simulink model "test_SimulinkMdl2_qLPVMPCbeta"  (R2023a)
settings: Solver=FixedStepAuto  StartTime=0.0  StopTime=400  FixedStep=DT  RelTol=1e-3
values from neighbouring files (symbols this model uses):
  DT = 0.008    [dataDLR.m]    (also in generateReport.m; initLPVParam.m; initWorkspace.m; runCalculateEvalCriteria.m)
  Lin_points : value not decoded    [DD_test.sldd]
undefined symbols (not defined in the file or in its folder): Rotor_Lambda
settings Model: DataDictionary=DD_test.sldd  ExtModeTrigMode=oneshot  Creator=Hazim Namik  LastModifiedBy=ditt_aj
settings SolverCC: AlgebraicLoopSolver=TrustRegion
settings DataIOCC: LimitDataPoints=on  SaveFormat=Array  ReturnWorkspaceOutputs=off
settings OptimizationCC: BlockReduction=off  BooleanDataType=off  LifeSpan=inf
settings DebuggingCC: SaveWithParameterizedLinksMsg=none  UnderspecifiedInitializationDetection=Classic  MergeDetectMultiDrivingBlocksExec=none  SignalResolutionControl=TryResolveAllWithWarning  UnconnectedInputMsg=warning  UnconnectedOutputMsg=warning  UnconnectedLineMsg=warning  SFUnexpectedBacktrackingDiag=warning  SFNoUnconditionalDefaultTransitionDiag=warning  SFExecutionAtInitializationDiag=none  ArithmeticOperatorsInVariantConditions=warning
settings HardwareCC: ProdBitPerPointer=32  ProdBitPerSizeT=32  ProdBitPerPtrDiffT=32  ProdLargestAtomicFloat=None  ProdIntDivRoundTo=Undefined  ProdEndianess=Unspecified  ProdWordSize=32  ProdHWDeviceType=32-bit Generic  TargetUnknown=on
settings ModelReferenceCC: EnableRefExpFcnMdlSchedulingChecks=on  PropagateSignalLabelsOutOfModel=off
settings SFSimCC: SimUseLocalCustomCode=off  CustomCodeUndefinedFunction=UseInterfaceOnly
settings RTWCC: RTWUseLocalCustomCode=off  DLArmComputeVersion=19.05
settings CodeAppCC: StateflowObjectComments=on
settings GRTTargetCC: TargetLangStandard=C89/C90 (ANSI)
settings ConfigComp: CovMetricSettings=dw  CovSaveCumulativeToWorkspaceVar=on  CovSaveSingleToWorkspaceVar=on  CovExternalEMLEnable=off

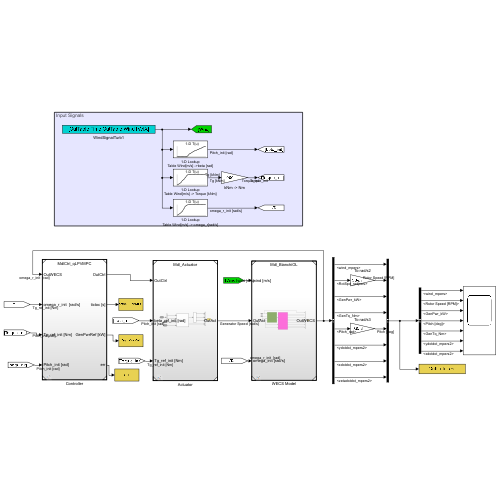
[thumbnail: Simulink's stored preview of the top-level diagram]
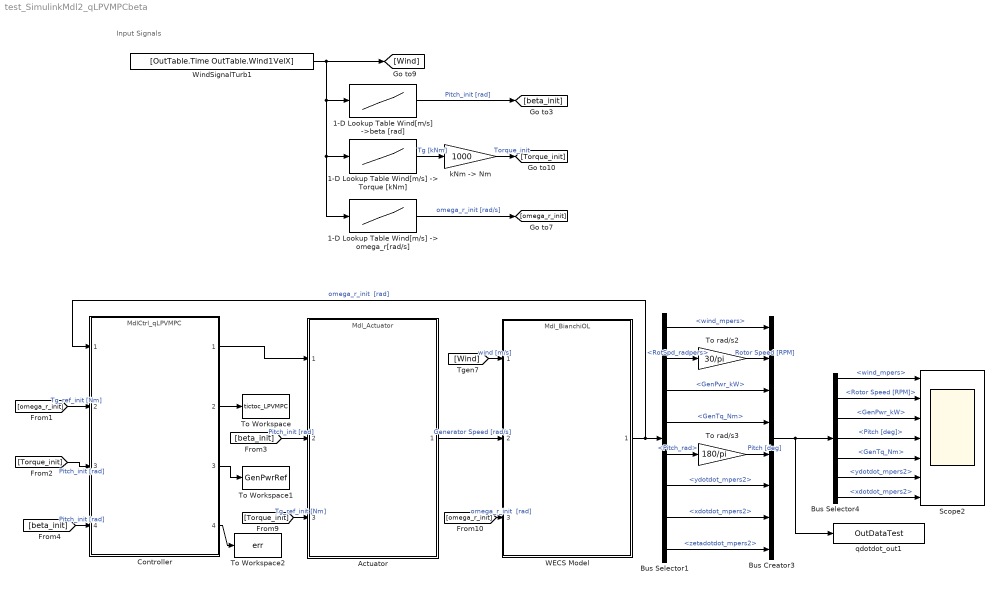
== system test_SimulinkMdl2_qLPVMPCbeta ==
  note: Input Signals
  "1-D Lookup Table Wind[m/s] -> Torque [kNm]" : Lookup_n-D  NumberOfTableDimensions=1  BreakpointsForDimension1=Lin_points.V  BreakpointsForDimension2=Rotor_Lambda  Table=Lin_points.Torque  InternalRulePriority=Speed  RndMeth=Simplest
  "1-D Lookup Table Wind[m/s] -> omega_r[rad/s]" : Lookup_n-D  NumberOfTableDimensions=1  BreakpointsForDimension1=Lin_points.V  BreakpointsForDimension2=Rotor_Lambda  Table=Lin_points.RSpeed  InternalRulePriority=Speed  RndMeth=Simplest
  1-D Lookup Table Wind[m/s] ->beta [rad] : Lookup_n-D  NumberOfTableDimensions=1  BreakpointsForDimension1=Lin_points.V  BreakpointsForDimension2=Rotor_Lambda  Table=Lin_points.Pitch  InternalRulePriority=Speed  RndMeth=Simplest
  Actuator : ModelReference  ModelNameDialog=Mdl_Actuator.slx  SimulationMode=Normal  ModelReferenceVersion=7.0
  Bus Creator3 : BusCreator  Inputs=8
  Bus Selector1 : BusSelector  OutputSignals=wind_mpers,RotSpd_radpers,GenPwr_kW,GenTq_Nm,Pitch_rad,ydotdot_mpers2,xdotdot_mpers2,zetadotdot_mpers2
  Bus Selector4 : BusSelector  OutputSignals=wind_mpers,Rotor Speed [RPM],GenPwr_kW,Pitch [deg],GenTq_Nm,ydotdot_mpers2,xdotdot_mpers2
  Controller : ModelReference  ModelNameDialog=MdlCtrl_qLPVMPC.slx  SimulationMode=Normal  ModelReferenceVersion=7.38
  Scope2 : Scope  NumInputPorts=7
      settings: Tag=Scope
  To Workspace : ToWorkspace  VariableName=tictoc_LPVMPC  SaveFormat=Timeseries  SampleTime=-1
  To Workspace1 : ToWorkspace  VariableName=GenPwrRef  SaveFormat=Timeseries  SampleTime=-1
  To Workspace2 : ToWorkspace  VariableName=err  SaveFormat=Timeseries  SampleTime=-1
  To rad/s2 : Gain  Gain=30/pi
  To rad/s3 : Gain  Gain=180/pi
  WECS Model : ModelReference  ModelNameDialog=Mdl_BianchiOL.slx  SimulationMode=Normal  ModelReferenceVersion=7.1
  WindSignalTurb1 : FromWorkspace  VariableName=[OutTable.Time OutTable.Wind1VelX]  SampleTime=DT  OutputAfterFinalValue=Holding final value
  "kNm -> Nm" : Gain  Gain=1000
  qdotdot_out1 : ToWorkspace  VariableName=OutDataTest  SampleTime=-1
  wires:
  [Torque_init] -> Controller/3  "Pitch_init [rad]"
  WindSignalTurb1/1 -> [Wind], "1-D Lookup Table Wind[m/s] -> omega_r[rad/s]"/1, "1-D Lookup Table Wind[m/s] -> Torque [kNm]"/1, 1-D Lookup Table Wind[m/s] ->beta [rad]/1
  "kNm -> Nm"/1 -> [Torque_init]  "Torque_init"
  [omega_r_init] -> Controller/2  "Tg_ref_init [Nm]"
  "1-D Lookup Table Wind[m/s] -> omega_r[rad/s]"/1 -> [omega_r_init]  "omega_r_init [rad/s]"
  [Wind] -> WECS Model/1  "wind [m/s]"
  1-D Lookup Table Wind[m/s] ->beta [rad]/1 -> [beta_init]  "Pitch_init [rad]"
  "1-D Lookup Table Wind[m/s] -> Torque [kNm]"/1 -> "kNm -> Nm"/1  "Tg [kNm]"
  [Torque_init] -> Actuator/3  "Tg_ref_init [Nm]"
  Actuator/1 -> WECS Model/2  "Generator Speed [rad/s]"
  [omega_r_init] -> WECS Model/3  "omega_r_init  [rad]"
  Controller/3 -> To Workspace1/1
  [beta_init] -> Actuator/2  "Pitch_init [rad]"
  Bus Selector1/5 -> To rad/s3/1  "<Pitch_rad>"
  To rad/s2/1 -> Bus Creator3/2  "Rotor Speed [RPM]"
  Bus Creator3/1 -> qdotdot_out1/1, Bus Selector4/1
  Bus Selector4/4 -> Scope2/4  "<Pitch [deg]>"
  Bus Selector4/7 -> Scope2/7  "<xdotdot_mpers2>"
  Bus Selector4/6 -> Scope2/6  "<ydotdot_mpers2>"
  Bus Selector4/1 -> Scope2/1  "<wind_mpers>"
  To rad/s3/1 -> Bus Creator3/5  "Pitch [deg]"
  Bus Selector4/5 -> Scope2/5  "<GenTq_Nm>"
  Bus Selector1/2 -> To rad/s2/1  "<RotSpd_radpers>"
  Bus Selector1/1 -> Bus Creator3/1  "<wind_mpers>"
  Bus Selector1/4 -> Bus Creator3/4  "<GenTq_Nm>"
  Bus Selector1/3 -> Bus Creator3/3  "<GenPwr_kW>"
  Bus Selector1/7 -> Bus Creator3/7  "<xdotdot_mpers2>"
  Bus Selector1/6 -> Bus Creator3/6  "<ydotdot_mpers2>"
  Bus Selector4/3 -> Scope2/3  "<GenPwr_kW>"
  Bus Selector4/2 -> Scope2/2  "<Rotor Speed [RPM]>"
  WECS Model/1 -> Controller/1, Bus Selector1/1  "omega_r_init  [rad]"
  [beta_init] -> Controller/4  "Pitch_init [rad]"
  Controller/1 -> Actuator/1
  Controller/2 -> To Workspace/1
  Controller/4 -> To Workspace2/1
  Bus Selector1/8 -> Bus Creator3/8  "<zetadotdot_mpers2>"
